simulink model "enr312_pendulum"  (R2026a)
settings: Solver=ode45  StopTime=P.stopTime  MaxStep=5e-4  RelTol=1e-6
values from neighbouring files (symbols this model uses):
  P = struct('exp', exp)    [enr312_simulink_params.m]    (also in run_enr312_simulink.m = enr312_simulink_params(e))
settings Model: Creator=odyssix  LastModifiedBy=odyssix

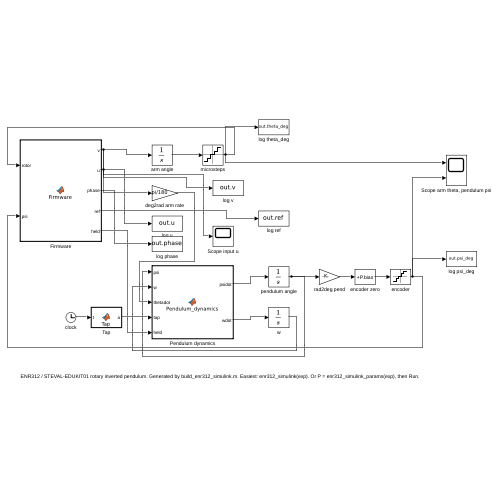
[thumbnail: Simulink's stored preview of the top-level diagram]
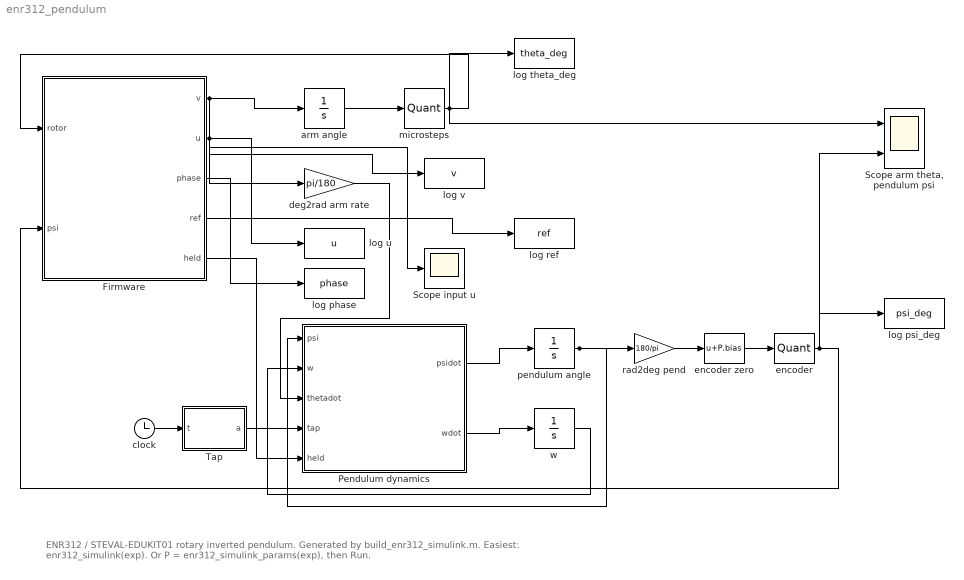
== system enr312_pendulum ==
  note: ENR312 / STEVAL-EDUKIT01 rotary inverted pendulum. Generated by build_enr312_simulink.m. Easiest: enr312_simulink(exp). Or P = enr312_simulink_params(exp), then Run.
  Firmware : MATLAB Function  TreatAsAtomicUnit=on
  Pendulum dynamics : MATLAB Function  TreatAsAtomicUnit=on
  "Scope arm theta, pendulum psi" : Scope  NumInputPorts=2
  Scope input u : Scope
  Tap : MATLAB Function  TreatAsAtomicUnit=on
  arm angle : Integrator
  clock : Clock
  deg2rad arm rate : Gain  Gain=pi/180
  encoder : Quantizer  QuantizationInterval=P.encDeg
  encoder zero : Bias  Bias=P.bias  SaturateOnIntegerOverflow=off
  log phase : ToWorkspace  VariableName=phase  SaveFormat=Timeseries  SampleTime=-1
  log psi_deg : ToWorkspace  VariableName=psi_deg  SaveFormat=Timeseries  SampleTime=-1
  log ref : ToWorkspace  VariableName=ref  SaveFormat=Timeseries  SampleTime=-1
  log theta_deg : ToWorkspace  VariableName=theta_deg  SaveFormat=Timeseries  SampleTime=-1
  log u : ToWorkspace  VariableName=u  SaveFormat=Timeseries  SampleTime=-1
  log v : ToWorkspace  VariableName=v  SaveFormat=Timeseries  SampleTime=-1
  microsteps : Quantizer  QuantizationInterval=P.stepDeg
  pendulum angle : Integrator  InitialCondition=P.psi0*pi/180
  rad2deg pend : Gain  Gain=180/pi
  w : Integrator
  wires:
  Firmware/1(v) -> arm angle/1, deg2rad arm rate/1, log v/1
  arm angle/1 -> microsteps/1
  microsteps/1 -> Firmware/1(rotor), log theta_deg/1, "Scope arm theta, pendulum psi"/1
  deg2rad arm rate/1 -> Pendulum dynamics/3(thetadot)
  pendulum angle/1 -> Pendulum dynamics/1(psi), rad2deg pend/1
  w/1 -> Pendulum dynamics/2(w)
  clock/1 -> Tap/1(t)
  Tap/1(a) -> Pendulum dynamics/4(tap)
  Firmware/5(held) -> Pendulum dynamics/5(held)
  Pendulum dynamics/1(psidot) -> pendulum angle/1
  Pendulum dynamics/2(wdot) -> w/1
  rad2deg pend/1 -> encoder zero/1
  encoder zero/1 -> encoder/1
  encoder/1 -> Firmware/2(psi), log psi_deg/1, "Scope arm theta, pendulum psi"/2
  Firmware/2(u) -> log u/1, Scope input u/1
  Firmware/3(phase) -> log phase/1
  Firmware/4(ref) -> log ref/1

== matlab function enr312_pendulum/Pendulum dynamics ==
  data: psi input; psidot output; w input; thetadot input; tap input; held input; wdot output; P parameter
function [psidot, wdot] = Pendulum_dynamics(psi, w, thetadot, tap, held, P)
% rigid pendulum on a rotating arm (docs/first_principles/ROTARY_PENDULUM_DYNAMICS.md, eq. 6)
% plus dry pivot friction, smoothed as c*tanh(psidot/width); all in rad.
% State w = psidot - wr2 cos(psi) thetadot removes the arm acceleration from the
% equation: a step in the arm velocity changes psidot by wr2 cos(psi) times the step.
if held > 0.5
    psidot = 0; wdot = 0; return;      % the hand holds it still
end
psidot = w + P.wr2 * cos(psi) * thetadot;
wdot = -P.wg2 * sin(psi) + thetadot^2 * sin(psi) * cos(psi) - P.gamma * psidot ...
       - P.coulomb * tanh(psidot / P.coulombWidth) + P.wr2 * sin(psi) * psidot * thetadot + tap;
end

== matlab function enr312_pendulum/Firmware ==
  settings: updateMethod=DISCRETE  sampleTime=P.Ts
  data: rotor input; v output; psi input; u output; phase output; ref output; held output; P parameter
function [v, u, phase, ref, held] = Firmware(rotor, psi, P)
% The firmware's control loop, one call per 2 ms tick (Enr312Firmware.m, a port of
% firmware/enr312/src). rotor: the arm in microsteps (deg); psi: the encoder (deg).
% v: arm velocity for the next tick (deg/s); u: plant input (deg/s^2); held: 1 while
% the operator's hand holds the pendulum at the start of an upright experiment.
coder.extrinsic('enr312_fw_tick');
persistent first
if isempty(first), first = true; end
v = 0; u = 0; phase = 0; ref = 0; held = 0;
[v, u, phase, ref, held] = enr312_fw_tick(first, rotor, psi, P);
first = false;
end

== matlab function enr312_pendulum/Tap ==
  data: t input; a output; P parameter
function a = Tap(t, P)
% a tap: P.tapRate deg/s added to the rate of the tilt from upright, spread over
% P.tapWidth s. The tilt from upright is 180 deg - psi.
a = 0;
if P.tapRate ~= 0 && t >= P.tapTime && t < P.tapTime + P.tapWidth
    a = -P.tapRate * pi / 180 / P.tapWidth;
end
end
